simulink model "Loop_Bandwidth_Noise_Suppression"  (R2025a)
settings: Solver=VariableStepAuto  StartTime=0.0  StopTime=500  RelTol=1e-3
libraries: simulink x4
settings Model: Creator=庞亚宸  LastModifiedBy=庞亚宸

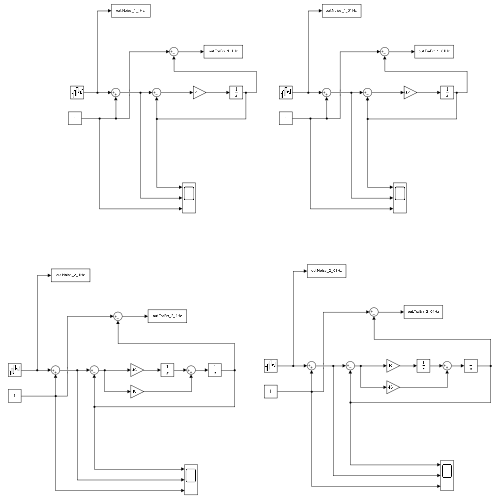
[thumbnail: Simulink's stored preview of the top-level diagram]
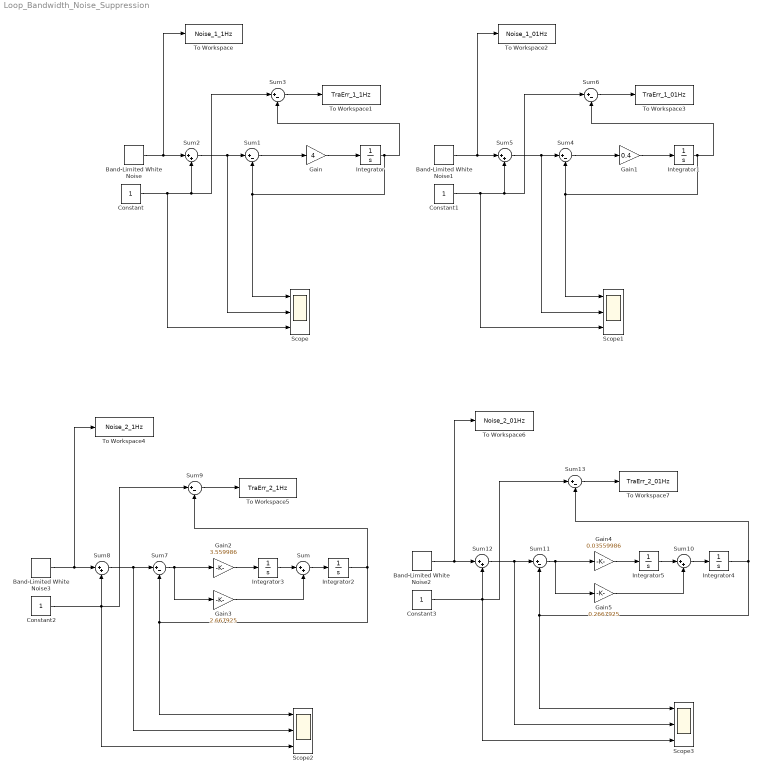
== system Loop_Bandwidth_Noise_Suppression ==
  Band-Limited White Noise{,1..3} (4 alike) : simulink/Sources/Band-Limited White Noise  Cov=[1]  Ts=0.01  seed=[23341]
  Constant{,1..3} (4 alike) : Constant
  Gain : Gain  Gain=4
  Gain1 : Gain  Gain=0.4
  Gain2 : Gain  Gain=3.559986
  Gain3 : Gain  Gain=2.667925
  Gain4 : Gain  Gain=0.03559986
  Gain5 : Gain  Gain=0.2667925
  Integrator{,1..5} (6 alike) : Integrator
  Scope{,1..3} (4 alike) : Scope  NumInputPorts=3
      Scope settings: ActiveDisplayYMinimum=-0.93963080728728676  ActiveDisplayYMaximum=2.6407729197115568
      Scope1 settings: ActiveDisplayYMinimum=-0.93963080728728676  ActiveDisplayYMaximum=2.6407729197115568
      Scope2 settings: ActiveDisplayYMinimum=-0.7962598709862958  ActiveDisplayYMaximum=2.6188896236694434  DataLoggingVariableName=ScopeData2
      Scope3 settings: ActiveDisplayYMinimum=-0.93963080728728676  ActiveDisplayYMaximum=2.6407729197115568  DataLoggingVariableName=ScopeData3
  Sum{,2,5,8,10,12} (6 alike) : Sum  Inputs=|++
  Sum{1,3..4,6..7,9,11,13} (8 alike) : Sum  Inputs=|+-
  To Workspace : ToWorkspace  VariableName=Noise_1_1Hz  SampleTime=0.01
  To Workspace1 : ToWorkspace  VariableName=TraErr_1_1Hz  SampleTime=0.01
  To Workspace2 : ToWorkspace  VariableName=Noise_1_01Hz  SampleTime=0.01
  To Workspace3 : ToWorkspace  VariableName=TraErr_1_01Hz  SampleTime=0.01
  To Workspace4 : ToWorkspace  VariableName=Noise_2_1Hz  SampleTime=0.01
  To Workspace5 : ToWorkspace  VariableName=TraErr_2_1Hz  SampleTime=0.01
  To Workspace6 : ToWorkspace  VariableName=Noise_2_01Hz  SampleTime=0.01
  To Workspace7 : ToWorkspace  VariableName=TraErr_2_01Hz  SampleTime=0.01
  wires:
  Integrator/1 -> Sum3/2, Sum1/2, Scope/1
  Sum1/1 -> Gain/1
  Gain/1 -> Integrator/1
  Band-Limited White Noise/1 -> To Workspace/1, Sum2/1
  Constant/1 -> Scope/3, Sum2/2, Sum3/1
  Sum2/1 -> Scope/2, Sum1/1
  Sum3/1 -> To Workspace1/1
  Sum5/1 -> Scope1/2, Sum4/1
  Constant1/1 -> Scope1/3, Sum5/2, Sum6/1
  Band-Limited White Noise1/1 -> To Workspace2/1, Sum5/1
  Sum4/1 -> Gain1/1
  Sum6/1 -> To Workspace3/1
  Gain1/1 -> Integrator1/1
  Integrator1/1 -> Sum6/2, Sum4/2, Scope1/1
  Sum/1 -> Integrator2/1
  Gain3/1 -> Sum/2
  Gain2/1 -> Integrator3/1
  Integrator3/1 -> Sum/1
  Sum7/1 -> Gain3/1, Gain2/1
  Integrator2/1 -> Sum9/2, Scope2/1, Sum7/2
  Sum8/1 -> Scope2/2, Sum7/1
  Band-Limited White Noise3/1 -> To Workspace4/1, Sum8/1
  Constant2/1 -> Sum9/1, Scope2/3, Sum8/2
  Sum9/1 -> To Workspace5/1
  Sum13/1 -> To Workspace7/1
  Integrator4/1 -> Sum13/2, Scope3/1, Sum11/2
  Sum11/1 -> Gain5/1, Gain4/1
  Gain4/1 -> Integrator5/1
  Integrator5/1 -> Sum10/1
  Sum10/1 -> Integrator4/1
  Band-Limited White Noise2/1 -> To Workspace6/1, Sum12/1
  Sum12/1 -> Scope3/2, Sum11/1
  Constant3/1 -> Sum13/1, Scope3/3, Sum12/2
  Gain5/1 -> Sum10/2
